simulink model "DCFastCharger"  (R2026b)
settings: Solver=ode23t  StopTime=simulation.simTime  MaxStep=1/(5*inverter.SwitchFrequency)  AbsTol=1e-3
PreLoadFcn:
  | run('DCFastChargerData.mlx');
undefined symbols (not defined in the file or in its folder): battery, inverter, rectifier
libraries: nesl_utility x34, fl_lib x22, ee_lib x14, eePwmGenerator x2, eeTransforms x2, batteryecm_lib x1, eeSinusoidalMeasurement x1, slpidlib x1, eePwmGeneratorThreeLevel x1, eePwmGeneratorTwoLevel x1, simulink_extras x1
(part 1 of 3)
settings Model: Creator=The MathWorks, Inc.  LastModifiedBy=patkruadamrong
settings SolverCC: AutoScaleAbsTol=off
settings DataIOCC: DSMLogging=off  ReturnWorkspaceOutputs=off  SaveState=on  SignalLogging=off
settings OptimizationCC: ReuseModelBlockBuffer=off
settings DebuggingCC: IgnoredZcDiagnostic=none
settings RTWCC: DLArmComputeVersion=19.05
settings SimscapeCC: SimscapeLogLimitData=off  SimscapeLogName=simlog_DCFastCharger  SimscapeLogSimulationStatistics=on  SimscapeLogType=all  SimscapeUseEnergyAccounting=off

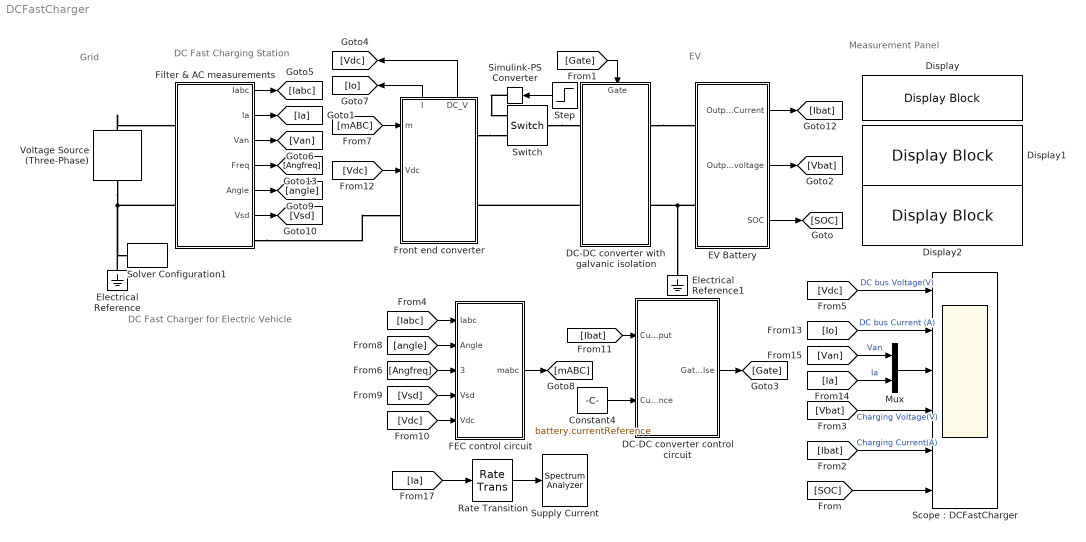
== system DCFastCharger ==
  note: Measurement Panel
  note: Grid
  note: DC Fast Charging Station
  note: EV
  note: DC Fast Charger for Electric Vehicle
  Constant4 : Constant  Value=battery.currentReference
  DC-DC converter with galvanic isolation : Subsystem
      settings: PortSchema="{\"entries\":[{\"content\":{\"sides\":[{\"content\":{\"connectorIds\":[\"LConn1\",\"LConn2\"]},\"type\":\"ConnectorPlacement.EquallySpacedRectSide\",\"uuid\":\"cdc417bd-b70c-4a8b-af35-4387024a7132\"},{\"content\":{\"connectorIds\":[\"RConn1\",\"RConn2\"],\"side\":\"RIGHT\"},\"type\":\"ConnectorPlacement.EquallySpacedRectSide\",\"uuid\":\"7ffe8d7a-a957-4278-941d-227fd05ae124\"},{\"content\":{\"connectorIds\":[\"In1\"],\"side\":\"TOP\"},\"type\":\"ConnectorPlacement.EquallySpacedRectSide\",\"uuid\":\"a7a81929-1a7a-4c69-b225-a78f4f2fe477\"}]},\"type\":\"ConnectorPlacement.EquallySpacedConnector\",\"uuid\":\"ce8dd18f-fb87-4936-99a6-3d248ca5aaa5\"}],\"packageUris\":[\"http://schema.mathworks.com/mf0/Connector/R2020b\"],\"version\":\"1.0\"}"
  DC-DC converter control circuit : Subsystem
  Display : DisplayBlock  Format=Integer  Transparency=1  GridColor=[0.502, 0.502, 0.502]  ShowGrid=off
  Display1 : DisplayBlock  Transparency=1  GridColor=[0.502, 0.502, 0.502]
  Display2 : DisplayBlock  Transparency=1  GridColor=[0.502, 0.502, 0.502]
  EV Battery : Subsystem
  Electrical Reference : fl_lib/Electrical/Electrical Elements/Electrical Reference
  Electrical Reference1 : fl_lib/Electrical/Electrical Elements/Electrical Reference
  FEC control circuit : Subsystem
  Filter & AC measurements : Subsystem
  Front end converter : Subsystem
      settings: PortSchema="{\"entries\":[{\"content\":{\"sides\":[{\"content\":{\"connectorIds\":[\"In1\",\"In2\",\"LConn1\"]},\"type\":\"ConnectorPlacement.EquallySpacedRectSide\",\"uuid\":\"e0050959-187d-4376-aad2-f8df21a08105\"},{\"content\":{\"connectorIds\":[\"RConn1\",\"RConn2\"],\"side\":\"RIGHT\"},\"type\":\"ConnectorPlacement.EquallySpacedRectSide\",\"uuid\":\"f7268924-358f-4021-b832-f47ce5e56f0e\"},{\"content\":{\"connectorIds\":[\"Out1\",\"Out2\"],\"side\":\"TOP\"},\"type\":\"ConnectorPlacement.EquallySpacedRectSide\",\"uuid\":\"ee33ccaf-ad48-493d-8220-739115e3c7e4\"}]},\"type\":\"ConnectorPlacement.EquallySpacedConnector\",\"uuid\":\"0bbfb8b2-bc26-491a-a2fb-5c6420aeb7c8\"}],\"packageUris\":[\"http://schema.mathworks.com/mf0/Connector/R2020b\"],\"version\":\"1.0\"}"
  Mux : Mux  Inputs=2
  Rate Transition : RateTransition  OutPortSampleTime=1/(10*rectifier.SwitchFrequency)
  "Scope : DCFastCharger" : Scope  NumInputPorts=6
      settings: TimeSpan=simulation.simTime  Title=FEC Output DC Voltage (V)  ActiveDisplayYMinimum=550.11802498602185  ActiveDisplayYMaximum=917.03777512580245  DataLoggingVariableName=ScopeData2
  Simulink-PS Converter : nesl_utility/Simulink-PS Converter  PhysicalDomain=network_engine_domain  SubClassName=ps_input  LeftPortType=input  RightPortType=output  PseudoPeriodic=off  Frequencies=[]  NoiseDistribution=none  NoiseParameters=[]  Unit=1  AffineConversion=off  FilteringAndDerivatives=provide  SimscapeFilterOrder=1  InputFilterTimeConstant=0.001  UdotUserProvided=0
  Solver Configuration1 : nesl_utility/Solver Configuration  PhysicalDomain=network_engine_domain  SubClassName=solver  LeftPortType=input  RightPortType=generic  Tones=[]  Harmonics=[]  SimulateNoise=off  Profile=off  UseLocalSampling=off  EnableSwitchedLinearOptims=on  FrequencyDomain=off  UseCCode=off  RelTol=0.001  AbsTol=1e-06  MinStep=1e-09  ToWorkspace=off  RevertToSquareIcSolve=off  NumHomotopyIterations=100  PhasorMode=off  PhasorModeNumHarmonics=1  ConsistencySolver=NEWTON_FTOL  CanonicalOrdering=UNORDERED  OptimizeIntermediates=UNOPTIMIZED  MulticoreSolverChoice=BACKWARD_EULER  IndexReductionMethod=DerivativeReplacement  DoDC=off  ResidualTolerance=1e-9  ConsistencyTolSource=GLOBAL  ConsistencyAbsTol=0.001  ConsistencyRelTol=0.001  ConsistencyTolFactor=0.001  UseLocalSolver=off  LocalSolverChoice=NE_PARTITIONING_ADVANCER  ResolveIndetEquations=on  FunctionEvalNumThread=1  LocalSolverSampleTime=1e-6  DoFixedCost=on  MaxNonlinIter=10  MaxModeIter=2  ComputeImpulses=off  ImpulseIterations=2  LinearAlgebra=auto  LinearAlgebraNumThread=0  EquationFormulation=NE_TIME_EF  DelaysMemoryBudget=1024  AutomaticFiltering=on  FilteringTimeConstant=0.001  PartitionStorageMethod=AS_NEEDED  PartitionMemoryBudget=1024  PartitionMethod=FAST  MultibodyUseLocalSolver=off  MultibodyLocalSolverChoice=ODE1  MultibodyLocalSolverSampleTime=0.001
  Step : Step  Time=0.02  SampleTime=0
  Supply Current : SpectrumAnalyzer  WindowPosition=[155.000000,395.000000,620.000000,438.000000,]  Visible=on  ScopeFrameLocation=window  SpectrumType=RMS  Method=Welch  SampleRate=100000  PlotAsTwoSidedSpectrum=off  FrequencyScale=Log  AxesScaling=Manual  RBWSource=Property  RBW=9  Span=50000  CenterFrequency=25000  StartFrequency=0  StopFrequency=50000  OverlapPercent=90  AveragingMethod=Running  SpectrumUnits=Vrms  YLimits=[-14.273478476221832523 128.46167495283401649]  ColorLimits=[0.0061790664803535039207 16.888204283875005274]  AllowFFTLengthLessThanSamplesPerUpdate=on
  Switch : fl_lib/Electrical/Electrical Elements/Switch  R_closed=0.01 Ohm  G_open=1e-8 1/Ohm  Threshold=0.5  i_specify=off  i_priority=None  i=0 A  i_nominal_specify=off  i_nominal_value=1  i_nominal_unit=A  v_specify=off  v_priority=None  v=0 V  v_nominal_specify=off  v_nominal_value=1  v_nominal_unit=V
  Voltage Source (Three-Phase) : ee_lib/Sources/Voltage Source (Three-Phase)  vline_rms=rectifier.ACVoltagePP V  shift=0 deg  freq=rectifier.SystemFrequency Hz  impedance_option=0  SShortCircuit=1e6 V*A  XR=15  R=0.01 Ohm  L=3.97e-4 H  harmonic_option=0  harmonic_orders=[5, 7, 11, 13]  harmonic_ratios=[.1, .1, .1, .1]  G_parasitic=0 1/Ohm  I_specify=off  I_priority=None  I=[ 0 0 0 ] A  I_nominal_specify=off  I_nominal_value=1  I_nominal_unit=A
  wires:
  Mux/1 -> "Scope : DCFastCharger"/3
  [Io] -> "Scope : DCFastCharger"/2  "DC bus Current (A)"
  [Vdc] -> "Scope : DCFastCharger"/1  "DC bus Voltage(V)"
  [Ia] -> Mux/2  "Ia"
  Filter & AC measurements/1(Iabc) -> [Iabc]
  Step/1 -> Simulink-PS Converter/1
  DC-DC converter control circuit/1(GatePulse) -> [Gate]
  [Gate] -> DC-DC converter with galvanic isolation/1(Gate)
  Constant4/1 -> DC-DC converter control circuit/2(CurrentReference)
  [Iabc] -> FEC control circuit/1(Iabc)
  [angle] -> FEC control circuit/2(Angle)
  [Angfreq] -> FEC control circuit/3(Angfreq)
  [Vsd] -> FEC control circuit/4(Vsd)
  [Vdc] -> FEC control circuit/5(Vdc)
  FEC control circuit/1(mabc) -> [mABC]
  [mABC] -> Front end converter/1(m)
  [Vdc] -> Front end converter/2(Vdc)
  Front end converter/1(I) -> [Io]
  EV Battery/1(Output Current) -> [Ibat]
  EV Battery/2(Output voltage) -> [Vbat]
  [Ibat] -> DC-DC converter control circuit/1(CurrentInput)
  [Vbat] -> "Scope : DCFastCharger"/4  "Charging Voltage(V)"
  [Ibat] -> "Scope : DCFastCharger"/5  "Charging Current(A)"
  Filter & AC measurements/2(Ia) -> [Ia]
  Filter & AC measurements/3(Van) -> [Van]
  Front end converter/2(DC_V) -> [Vdc]
  Filter & AC measurements/4(Freq) -> [Angfreq]
  Filter & AC measurements/5(Angle) -> [angle]
  Filter & AC measurements/6(Vsd) -> [Vsd]
  EV Battery/3(SOC) -> [SOC]
  [SOC] -> "Scope : DCFastCharger"/6
  [Van] -> Mux/1  "Van"
  Rate Transition/1 -> Supply Current/1
  [Ia] -> Rate Transition/1
  connections:
  Simulink-PS Converter/RConn1 -- Switch/RConn1
  Voltage Source (Three-Phase)/RConn1 -- Filter & AC measurements/LConn1
  Switch/LConn1 -- DC-DC converter with galvanic isolation/LConn1
  DC-DC converter with galvanic isolation/LConn2 -- Front end converter/RConn2
  Voltage Source (Three-Phase)/LConn1 -- Electrical Reference/LConn1 -- Solver Configuration1/RConn1 -- Filter & AC measurements/LConn2
  Filter & AC measurements/RConn1 -- Front end converter/LConn1
  EV Battery/LConn2 -- DC-DC converter with galvanic isolation/RConn2 -- Electrical Reference1/LConn1
  DC-DC converter with galvanic isolation/RConn1 -- EV Battery/LConn1
  Front end converter/RConn1 -- Switch/RConn2

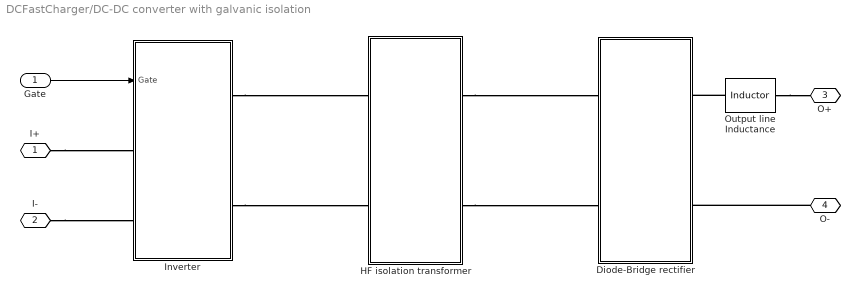
== system DCFastCharger/DC-DC converter with galvanic isolation ==
  Gate : Inport
  Diode-Bridge rectifier : Subsystem
  HF isolation transformer : Subsystem
  Inverter : Subsystem
  Output line Inductance : ee_lib/Passive/Inductor  l=battery.inductance H  enable_L_tol=0  L_tol=20  tol_distribution=1  nSigma=4  r=0 Ohm  g=1e-9 1/Ohm  enable_operating_limits=0  operating_limit_action=2  max_working_current=1 A  power_rating=1 W  i_L_specify=off  i_L_priority=High  i_L=80 A  i_L_nominal_specify=off  i_L_nominal_value=1  i_L_nominal_unit=A
  I+ : PMIOPort  Side=Left
  I- : PMIOPort  Port=2  Side=Left
  O+ : PMIOPort  Port=3  Side=Right
  O- : PMIOPort  Port=4  Side=Right
  wires:
  Gate/1 -> Inverter/1(Gate)
  connections:
  Inverter/RConn2 -- HF isolation transformer/LConn2
  O-/RConn1 -- Diode-Bridge rectifier/RConn2
  Inverter/RConn1 -- HF isolation transformer/LConn1
  HF isolation transformer/RConn1 -- Diode-Bridge rectifier/LConn1
  HF isolation transformer/RConn2 -- Diode-Bridge rectifier/LConn2
  I+/RConn1 -- Inverter/LConn1
  I-/RConn1 -- Inverter/LConn2
  Output line Inductance/RConn1 -- O+/RConn1
  Output line Inductance/LConn1 -- Diode-Bridge rectifier/RConn1

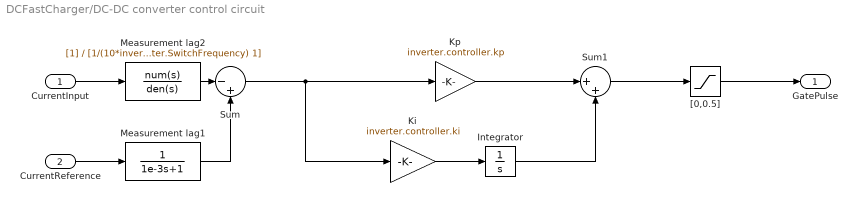
== system DCFastCharger/DC-DC converter control circuit ==
  CurrentInput : Inport
  CurrentReference : Inport  Port=2
  Integrator : Integrator  LimitOutput=on  UpperSaturationLimit=3  LowerSaturationLimit=-3
  Ki : Gain  Gain=inverter.controller.ki
  Kp : Gain  Gain=inverter.controller.kp
  Measurement lag1 : TransferFcn  Denominator=[1e-3 1]
  Measurement lag2 : TransferFcn  Denominator=[1/(10*inverter.SwitchFrequency) 1]
  Sum : Sum  Inputs=|-+
  Sum1 : Sum  Inputs=|++  InputSameDT=on  SaturateOnIntegerOverflow=on  OutDataTypeStr=Inherit: Same as first input
  "[0,0.5]" : Saturate  LowerLimit=0
  GatePulse : Outport
  wires:
  Sum/1 -> Ki/1, Kp/1
  Sum1/1 -> "[0,0.5]"/1
  "[0,0.5]"/1 -> GatePulse/1
  Kp/1 -> Sum1/1
  Ki/1 -> Integrator/1
  Integrator/1 -> Sum1/2
  Measurement lag2/1 -> Sum/1
  Measurement lag1/1 -> Sum/2
  CurrentReference/1 -> Measurement lag1/1
  CurrentInput/1 -> Measurement lag2/1

== system DCFastCharger/EV Battery ==
  EV Battery : Subsystem
      settings: PortSchema="{\"entries\":[{\"content\":{\"sides\":[{\"content\":{\"connectorIds\":[]},\"type\":\"ConnectorPlacement.EquallySpacedRectSide\",\"uuid\":\"8e1978f5-f19b-407a-84fd-c941bccecdad\"},{\"content\":{\"connectorIds\":[],\"side\":\"RIGHT\"},\"type\":\"ConnectorPlacement.EquallySpacedRectSide\",\"uuid\":\"fb49f29d-d34c-48f8-a58f-9f92c5d477c5\"},{\"content\":{\"connectorIds\":[\"LConn1\"],\"side\":\"TOP\"},\"type\":\"ConnectorPlacement.EquallySpacedRectSide\",\"uuid\":\"6762467a-e296-4691-a6dd-75c21ebdcdad\"},{\"content\":{\"connectorIds\":[\"Out1\",\"RConn1\"],\"side\":\"BOTTOM\"},\"type\":\"ConnectorPlacement.EquallySpacedRectSide\",\"uuid\":\"82209aad-7084-4f05-b357-bb8919115a4c\"}]},\"type\":\"ConnectorPlacement.EquallySpacedConnector\",\"uuid\":\"7c4645ca-e004-4a10-a314-5de950045894\"}],\"packageUris\":[\"http://schema.mathworks.com/mf0/Connector/R2020b\"],\"version\":\"1.0\"}"
  i : Subsystem
  v : Subsystem
  + : PMIOPort  Side=Left
  - : PMIOPort  Port=2  Side=Left
  Output Current : Outport
  Output voltage : Outport  Port=2
  SOC : Outport  Port=3
  wires:
  i/1(I) -> Output Current/1  "DC"
  v/1(V) -> Output voltage/1  "V"
  EV Battery/1(SOC) -> SOC/1
  connections:
  i/LConn1 -- +/RConn1
  -/RConn1 -- v/LConn1 -- EV Battery/RConn1
  i/RConn1 -- EV Battery/LConn1 -- v/RConn1

== system DCFastCharger/FEC control circuit ==
  Iabc : Inport
  Angle : Inport  Port=2
  Angfreq : Inport  Port=3
  Vsd : Inport  Port=4
  Vdc : Inport  Port=5
  Controller : Subsystem
  Modulation Signal : Subsystem
  mabc : Outport
  wires:
  Controller/1(Vd) -> Modulation Signal/1(Vd)
  Modulation Signal/1(mabc) -> mabc/1
  Controller/2(Vq) -> Modulation Signal/2(Vq)
  Vsd/1 -> Controller/4(Vsd)
  Iabc/1 -> Controller/1(Iabc)
  Vdc/1 -> Controller/5(Vdc)
  Angle/1 -> Modulation Signal/3(Angle), Controller/2(Angle)
  Angfreq/1 -> Controller/3(Angfreq)

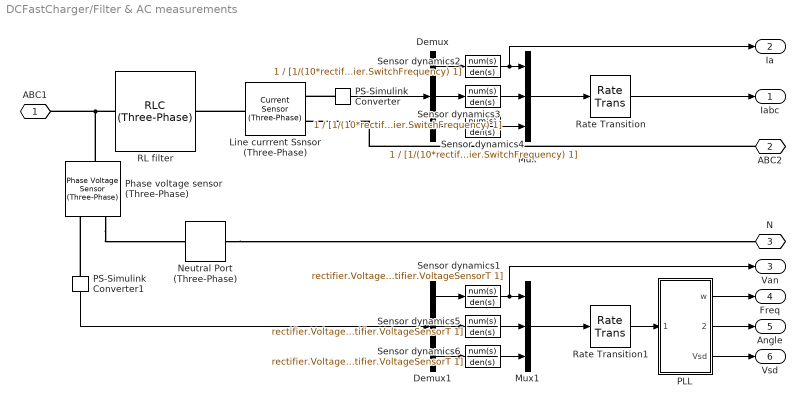
== system DCFastCharger/Filter & AC measurements ==
  Demux : Demux  Outputs=3
  Demux1 : Demux  Outputs=3
  Line currrent Ssnsor (Three-Phase) : ee_lib/Sensors & Transducers/Current Sensor (Three-Phase)  port_option=ee.enum.threePhasePort.composite
  Mux : Mux  Inputs=3
  Mux1 : Mux  Inputs=3
  Neutral Port (Three-Phase) : ee_lib/Connectors & References/Neutral Port (Three-Phase)  port_option=ee.enum.threePhasePort.composite  G_parasitic=1e-12 1/Ohm
  PLL : Subsystem
  PS-Simulink Converter : nesl_utility/PS-Simulink Converter  PhysicalDomain=network_engine_domain  SubClassName=ps_output  LeftPortType=input  RightPortType=output  PseudoPeriodic=off  Frequencies=[]  VectorFormat=1-D array  Unit=inherit  AffineConversion=off
  PS-Simulink Converter1 : nesl_utility/PS-Simulink Converter  PhysicalDomain=network_engine_domain  SubClassName=ps_output  LeftPortType=input  RightPortType=output  PseudoPeriodic=off  Frequencies=[]  VectorFormat=1-D array  Unit=inherit  AffineConversion=off
  Phase voltage sensor (Three-Phase) : ee_lib/Sensors & Transducers/Phase Voltage Sensor (Three-Phase)  port_option=ee.enum.threePhasePort.composite
  RL filter : ee_lib/Passive/RLC Assemblies/RLC (Three-Phase)  port_option=ee.enum.threePhasePort.composite  component_structure=ee.enum.rlc.structure.SeriesRL  R=rectifier.lineResistance Ohm  L=rectifier.lineInductance H  C=1e-6 F  R_parasitic=1e-6 Ohm  G_parasitic=1e-6 1/Ohm  IL_specify=on  IL_priority=High  IL=[0, 0, 0] A  IL_nominal_specify=off  IL_nominal_value=1  IL_nominal_unit=A  VC_specify=on  VC_priority=High  VC=[0, 0, 0] V  VC_nominal_specify=off  VC_nominal_value=1  VC_nominal_unit=V
  Rate Transition : RateTransition  OutPortSampleTime=1/(10*rectifier.SwitchFrequency)
  Rate Transition1 : RateTransition  OutPortSampleTime=rectifier.VoltageSensorT
  Sensor dynamics1 : TransferFcn  Numerator=rectifier.VoltageSensorG  Denominator=[rectifier.VoltageSensorT 1]
  Sensor dynamics2 : TransferFcn  Numerator=1  Denominator=[1/(10*rectifier.SwitchFrequency) 1]
  Sensor dynamics3 : TransferFcn  Numerator=1  Denominator=[1/(10*rectifier.SwitchFrequency) 1]
  Sensor dynamics4 : TransferFcn  Numerator=1  Denominator=[1/(10*rectifier.SwitchFrequency) 1]
  Sensor dynamics5 : TransferFcn  Numerator=rectifier.VoltageSensorG  Denominator=[rectifier.VoltageSensorT 1]
  Sensor dynamics6 : TransferFcn  Numerator=rectifier.VoltageSensorG  Denominator=[rectifier.VoltageSensorT 1]
  ABC1 : PMIOPort  Side=Left
  ABC2 : PMIOPort  Port=2  Side=Right
  N : PMIOPort  Port=3  Side=Left
  Iabc : Outport
  Ia : Outport  Port=2
  Van : Outport  Port=3
  Freq : Outport  Port=4
  Angle : Outport  Port=5
  Vsd : Outport  Port=6
  wires:
  Mux/1 -> Rate Transition/1
  Mux1/1 -> Rate Transition1/1
  PLL/3(Vsd) -> Vsd/1
  PLL/1(w) -> Freq/1
  PLL/2(angle) -> Angle/1
  Sensor dynamics4/1 -> Mux/3
  Demux/2 -> Sensor dynamics3/1
  Demux/3 -> Sensor dynamics4/1
  Demux/1 -> Sensor dynamics2/1
  Sensor dynamics2/1 -> Ia/1, Mux/1
  Sensor dynamics3/1 -> Mux/2
  Sensor dynamics6/1 -> Mux1/3
  Demux1/2 -> Sensor dynamics5/1
  Demux1/3 -> Sensor dynamics6/1
  Demux1/1 -> Sensor dynamics1/1
  Sensor dynamics1/1 -> Van/1, Mux1/1
  Sensor dynamics5/1 -> Mux1/2
  PS-Simulink Converter/1 -> Demux/1
  PS-Simulink Converter1/1 -> Demux1/1
  Rate Transition/1 -> Iabc/1
  Rate Transition1/1 -> PLL/1(Vabc)
  connections:
  Line currrent Ssnsor (Three-Phase)/LConn1 -- RL filter/RConn1
  ABC2/RConn1 -- Line currrent Ssnsor (Three-Phase)/RConn2
  PS-Simulink Converter/LConn1 -- Line currrent Ssnsor (Three-Phase)/RConn1
  PS-Simulink Converter1/LConn1 -- Phase voltage sensor (Three-Phase)/RConn1
  RL filter/LConn1 -- ABC1/RConn1 -- Phase voltage sensor (Three-Phase)/LConn1
  Neutral Port (Three-Phase)/RConn1 -- N/RConn1
  Phase voltage sensor (Three-Phase)/RConn2 -- Neutral Port (Three-Phase)/LConn1

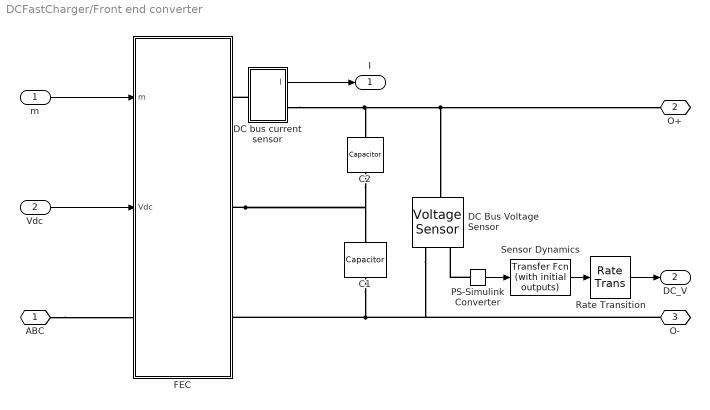
== system DCFastCharger/Front end converter ==
  m : Inport
  Vdc : Inport  Port=2
  C1 : fl_lib/Electrical/Electrical Elements/Capacitor  c=rectifier.OutputCapacitance*2 F  r=0.1e-3 Ohm  g=0 1/Ohm  i_specify=off  i_priority=High  i=0 A  i_nominal_specify=off  i_nominal_value=1  i_nominal_unit=A  v_specify=off  v_priority=High  v=0 V  v_nominal_specify=off  v_nominal_value=1  v_nominal_unit=V  vc_specify=on  vc_priority=High  vc=(rectifier.ACVoltagePP*1.414)/2*1.5 V  vc_nominal_specify=off  vc_nominal_value=1  vc_nominal_unit=V
  C2 : fl_lib/Electrical/Electrical Elements/Capacitor  c=rectifier.OutputCapacitance*2 F  r=0.1e-3 Ohm  g=0 1/Ohm  i_specify=off  i_priority=High  i=0 A  i_nominal_specify=off  i_nominal_value=1  i_nominal_unit=A  v_specify=off  v_priority=High  v=0 V  v_nominal_specify=off  v_nominal_value=1  v_nominal_unit=V  vc_specify=on  vc_priority=High  vc=(rectifier.ACVoltagePP*1.414)/2*1.5 V  vc_nominal_specify=off  vc_nominal_value=1  vc_nominal_unit=V
  DC Bus Voltage Sensor : fl_lib/Electrical/Electrical Sensors/Voltage Sensor
  DC bus current sensor : Subsystem
  FEC : Subsystem  Variant=on  VariantControl=Variant1
  PS-Simulink Converter : nesl_utility/PS-Simulink Converter  PhysicalDomain=network_engine_domain  SubClassName=ps_output  LeftPortType=input  RightPortType=output  PseudoPeriodic=off  Frequencies=[]  VectorFormat=1-D array  Unit=inherit  AffineConversion=off
  Rate Transition : RateTransition  OutPortSampleTime=rectifier.VoltageSensorT
  Sensor Dynamics : simulink_extras/Additional Linear/Transfer Fcn (with initial outputs)  N=rectifier.VoltageSensorG  D=[rectifier.VoltageSensorT 1]  Y0=rectifier.ACVoltagePP*1.414  U0=rectifier.ACVoltagePP*1.414
  ABC : PMIOPort  Side=Left
  O+ : PMIOPort  Port=2  Side=Right
  O- : PMIOPort  Port=3  Side=Right
  I : Outport
  DC_V : Outport  Port=2
  wires:
  m/1 -> FEC/1(m)
  Vdc/1 -> FEC/2(Vdc)
  DC bus current sensor/1(I) -> I/1
  Sensor Dynamics/1 -> Rate Transition/1
  PS-Simulink Converter/1 -> Sensor Dynamics/1
  Rate Transition/1 -> DC_V/1
  connections:
  ABC/RConn1 -- FEC/LConn1
  C1/RConn1 -- O-/RConn1 -- DC Bus Voltage Sensor/RConn2 -- FEC/RConn3
  FEC/RConn2 -- C1/LConn1 -- C2/RConn1
  DC bus current sensor/LConn1 -- FEC/RConn1
  PS-Simulink Converter/LConn1 -- DC Bus Voltage Sensor/RConn1
  DC bus current sensor/RConn1 -- O+/RConn1 -- DC Bus Voltage Sensor/LConn1 -- C2/LConn1

== system DCFastCharger/DC-DC converter with galvanic isolation/Diode-Bridge rectifier ==
  Diode{1..4} (4 alike) : fl_lib/Electrical/Electrical Elements/Diode  Vf=0.6 V  Ron=0.01 Ohm  Goff=1e-8 1/Ohm  i_specify=off  i_priority=None  i=0 A  i_nominal_specify=off  i_nominal_value=1  i_nominal_unit=A  v_specify=off  v_priority=None  v=0 V  v_nominal_specify=off  v_nominal_value=1  v_nominal_unit=V
  + : PMIOPort  Side=Right
  P : PMIOPort  Port=2  Side=Left
  - : PMIOPort  Port=3  Side=Right
  N : PMIOPort  Port=4  Side=Left
  connections:
  Diode4/RConn1 -- Diode2/RConn1 -- +/RConn1
  Diode1/LConn1 -- Diode3/LConn1 -- -/RConn1
  Diode4/LConn1 -- Diode1/RConn1 -- P/RConn1
  Diode3/RConn1 -- N/RConn1 -- Diode2/LConn1

== system DCFastCharger/DC-DC converter with galvanic isolation/HF isolation transformer ==
  Ideal Transformer : fl_lib/Electrical/Electrical Elements/Ideal Transformer  n=transformer.windingFactor  i1_specify=off  i1_priority=None  i1=0 A  i1_nominal_specify=off  i1_nominal_value=1  i1_nominal_unit=A  v1_specify=off  v1_priority=None  v1=0 V  v1_nominal_specify=off  v1_nominal_value=1  v1_nominal_unit=V  i2_specify=off  i2_priority=None  i2=0 A  i2_nominal_specify=off  i2_nominal_value=1  i2_nominal_unit=A  v2_specify=off  v2_priority=None  v2=0 V  v2_nominal_specify=off  v2_nominal_value=1  v2_nominal_unit=V
  Magnetizing Inductance : ee_lib/Passive/Inductor  l=transformer.magnetizingL H  enable_L_tol=0  L_tol=20  tol_distribution=1  nSigma=4  r=0 Ohm  g=1e-9 1/Ohm  enable_operating_limits=0  operating_limit_action=2  max_working_current=1 A  power_rating=1 W  i_L_specify=off  i_L_priority=High  i_L=0 A  i_L_nominal_specify=off  i_L_nominal_value=1  i_L_nominal_unit=A
  1+ : PMIOPort  Side=Left
  1- : PMIOPort  Port=2  Side=Left
  2+ : PMIOPort  Port=3  Side=Right
  2- : PMIOPort  Port=4  Side=Right
  connections:
  Ideal Transformer/RConn2 -- 2-/RConn1
  Ideal Transformer/LConn2 -- Magnetizing Inductance/RConn1 -- 1-/RConn1
  Ideal Transformer/LConn1 -- 1+/RConn1 -- Magnetizing Inductance/LConn1
  Ideal Transformer/RConn1 -- 2+/RConn1

== system DCFastCharger/DC-DC converter with galvanic isolation/Inverter ==
  Gate : Inport
  Four-Quadrant Chopper : ee_lib/Semiconductors & Converters/Converters/Four-Quadrant Chopper  fidelity_option=ee.enum.converters.fidelity.detailed  device_type=ee.enum.converters.switchingdevice.ideal  showThermalPort=false  Vgt=1 V  Vgt_off=-1 V  Ih=1 A  Vf=0.8 V  Ron=0.001 Ohm  Rds=0.001 Ohm  Goff=1e-5 1/Ohm  Vth=0.8 V  K=0  Eon_scalar=22.86e-3 J  Eoff_scalar=17.14e-3 J  Eoff_natural_commutation=10e-3 J  Voff=300 V  Iout_scalar=600 A  onCurrentMeasDelay=0 s  useCurrentFromPreviousCycle=false  useVoltageFromPreviousCycle=false  diode_param=ee.enum.converters.protectiondiode.nodynamics  diode_Vf=0.8 V  diode_Ron=0.001 Ohm  diode_Goff=1e-5 1/Ohm  diode_C=50 nF  diode_iRM=-235 A  diode_iF=300 A  diode_idot=-50 A/us  diode_trr_param=ee.enum.converters.diodetrr.trr_factor  diode_trr_factor=3  diode_trr=15 us  diode_Qrr=1500 s*uA  diode_rec_loss_model=ee.enum.diode.reverseRecoveryModel.fixed  diode_ErecVal=0 J  diode_scaleWithIandV=false  diode_ErecMat=zeros(2, 3) J  diode_TjrecVec=[298.15, 398.15] K  diode_IfrecVec=[.1, 1, 10] A  diode_IrecVal=10 A  diode_VrecVal=10 V  diode_tFilter=1 / 1000 / 100 s  thermal_network_parameterization=ee.enum.thermalNetworkTopology.external  Rth=[.08, .5] K/W  Rth_Cauer=[.08, .1, .5] K/W  Rth_Foster=[.08, .14, .22, .16] K/W  thermal_mass_parameterization=ee.enum.thermalNetwork.timeconstant  thermal_mass=[.01, .5] J/K  thermal_mass_Cauer=[.01, .1, .5] J/K  thermal_mass_Foster=[.001, .005, .05, .5] J/K  thermal_time_constant=[.001, .2] s  thermal_time_constant_Cauer=[.001, .1, .2] s  thermal_time_constant_Foster=[7e-05, .0007, .01, .08] s  thermal_mass_initial_temperatures=[25, 25] degC  thermal_mass_initial_temperatures_Cauer=[25, 25, 25] degC  junction_thermal_mass=0.01 J/K  Tvec_initial_Foster=[25, 25, 25, 25] degC  snubber_type=ee.enum.converters.snubber.exclude  Cs=1e-7 F  Rs=0.1 Ohm
  Gate drive : Subsystem
  P : PMIOPort  Side=Right
  + : PMIOPort  Port=2  Side=Left
  N : PMIOPort  Port=3  Side=Right
  - : PMIOPort  Port=4  Side=Left
  wires:
  Gate/1 -> Gate drive/1(Gate)
  connections:
  -/RConn1 -- Four-Quadrant Chopper/LConn3
  +/RConn1 -- Four-Quadrant Chopper/LConn2
  P/RConn1 -- Four-Quadrant Chopper/RConn1
  Four-Quadrant Chopper/RConn2 -- N/RConn1
  Gate drive/RConn1 -- Four-Quadrant Chopper/LConn1
